simulink model "lab23"  (R2025b)
settings: Solver=VariableStepAuto  StartTime=0.0  StopTime=10.0  RelTol=1e-3
undefined symbols (not defined in the file): A, B, Ds, Dt, Es, Et, kappa1, Keta, mb, T
settings Model: Creator=Nickolay  LastModifiedBy=Nickolay

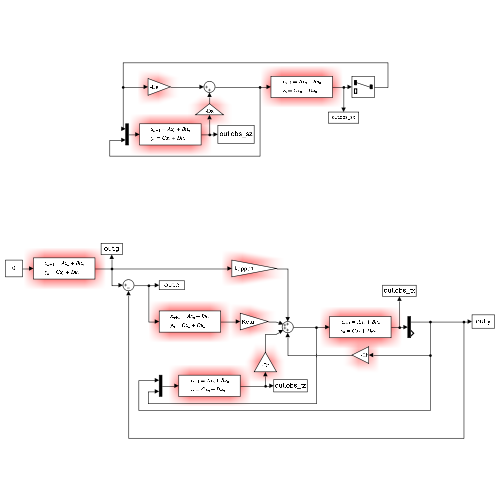
[thumbnail: Simulink's stored preview of the top-level diagram]
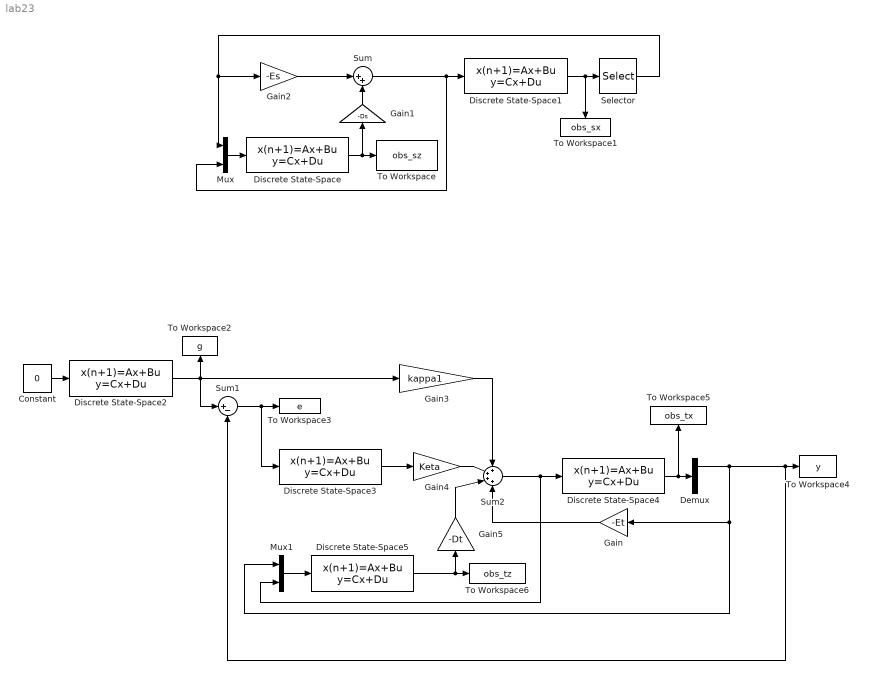
== system lab23 ==
  Constant : Constant  Value=0
  Demux : Demux  Outputs=2
  Discrete State-Space : DiscreteStateSpace  A=0  B=[1 mb]  D=[0 0]  SampleTime=T
  Discrete State-Space1 : DiscreteStateSpace  A=A  B=B  C=eye(2)  D=zeros(2,1)  InitialCondition=[1; 0]  SampleTime=T
  Discrete State-Space2 : DiscreteStateSpace  B=0  D=0  InitialCondition=2.8  SampleTime=T
  Discrete State-Space3 : DiscreteStateSpace  D=0  SampleTime=T
  Discrete State-Space4 : DiscreteStateSpace  A=A  B=B  C=eye(2)  D=[0; 0]  InitialCondition=[1; 0]  SampleTime=T
  Discrete State-Space5 : DiscreteStateSpace  A=0  B=[1 mb]  D=[0 0]  SampleTime=T
  Gain : Gain  Gain=-Et
  Gain1 : Gain  Gain=-Ds
  Gain2 : Gain  Gain=-Es
  Gain3 : Gain  Gain=kappa1
  Gain4 : Gain  Gain=Keta
  Gain5 : Gain  Gain=-Dt
  Mux : Mux  Inputs=2
  Mux1 : Mux  Inputs=2
  Selector : Selector  InputPortWidth=2  IndexOptions=Index vector (dialog)  Indices=1  OutputSizes=1
  Sum : Sum  Inputs=|++
  Sum1 : Sum  Inputs=|+-
  Sum2 : Sum  Inputs=++++
  To Workspace : ToWorkspace  VariableName=obs_sz  SaveFormat=Timeseries  SampleTime=-1
  To Workspace1 : ToWorkspace  VariableName=obs_sx  SaveFormat=Timeseries  SampleTime=-1
  To Workspace2 : ToWorkspace  VariableName=g  SaveFormat=Timeseries  SampleTime=-1
  To Workspace3 : ToWorkspace  VariableName=e  SaveFormat=Timeseries  SampleTime=-1
  To Workspace4 : ToWorkspace  VariableName=y  SaveFormat=Timeseries  SampleTime=-1
  To Workspace5 : ToWorkspace  VariableName=obs_tx  SaveFormat=Timeseries  SampleTime=-1
  To Workspace6 : ToWorkspace  VariableName=obs_tz  SaveFormat=Timeseries  SampleTime=-1
  wires:
  Mux/1 -> Discrete State-Space/1
  Discrete State-Space/1 -> Gain1/1, To Workspace/1
  Gain1/1 -> Sum/2
  Gain2/1 -> Sum/1
  Sum/1 -> Discrete State-Space1/1, Mux/2
  Discrete State-Space1/1 -> To Workspace1/1, Selector/1
  Selector/1 -> Mux/1, Gain2/1
  Demux/1 -> Mux1/1, Gain/1, Sum1/2, To Workspace4/1
  Gain4/1 -> Sum2/2
  Discrete State-Space3/1 -> Gain4/1
  Discrete State-Space4/1 -> To Workspace5/1, Demux/1
  Discrete State-Space2/1 -> To Workspace2/1, Gain3/1, Sum1/1
  Sum1/1 -> Discrete State-Space3/1, To Workspace3/1
  Constant/1 -> Discrete State-Space2/1
  Gain3/1 -> Sum2/1
  Sum2/1 -> Mux1/2, Discrete State-Space4/1
  Gain/1 -> Sum2/4
  Mux1/1 -> Discrete State-Space5/1
  Discrete State-Space5/1 -> Gain5/1, To Workspace6/1
  Gain5/1 -> Sum2/3
